simulink model "kubik_building_model"  (R2025a)
settings: Solver=ode45  StartTime=0.0  StopTime=86400  RelTol=1e-3
settings Model: Creator=Hp  LastModifiedBy=Hp

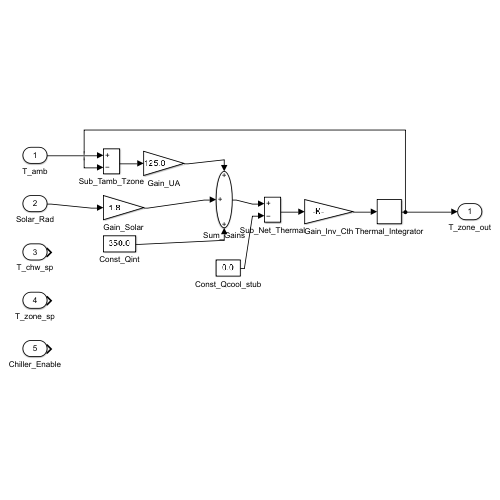
[thumbnail: Simulink's stored preview of the top-level diagram]
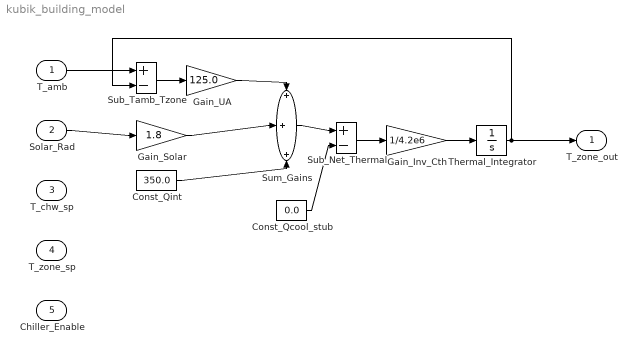
== system kubik_building_model ==
  T_amb : Inport
  Solar_Rad : Inport  Port=2
  T_chw_sp : Inport  Port=3
  T_zone_sp : Inport  Port=4
  Chiller_Enable : Inport  Port=5
  Const_Qcool_stub : Constant  Value=0.0
  Const_Qint : Constant  Value=350.0
  Gain_Inv_Cth : Gain  Gain=1/4.2e6
  Gain_Solar : Gain  Gain=1.8
  Gain_UA : Gain  Gain=125.0
  Sub_Net_Thermal : Sum  Inputs=+-
  Sub_Tamb_Tzone : Sum  Inputs=+-
  Sum_Gains : Sum  Inputs=+++
  Thermal_Integrator : Integrator  InitialCondition=24.2
  T_zone_out : Outport
  wires:
  T_amb/1 -> Sub_Tamb_Tzone/1
  Sub_Tamb_Tzone/1 -> Gain_UA/1
  Solar_Rad/1 -> Gain_Solar/1
  Gain_UA/1 -> Sum_Gains/1
  Gain_Solar/1 -> Sum_Gains/2
  Const_Qint/1 -> Sum_Gains/3
  Sum_Gains/1 -> Sub_Net_Thermal/1
  Gain_Inv_Cth/1 -> Thermal_Integrator/1
  Sub_Net_Thermal/1 -> Gain_Inv_Cth/1
  Thermal_Integrator/1 -> T_zone_out/1, Sub_Tamb_Tzone/2
  Const_Qcool_stub/1 -> Sub_Net_Thermal/2
